simulink library "Autonomous_lib"  (R2023b)
settings: Solver=VariableStepAuto  StartTime=0.0  StopTime=10.0  RelTol=1e-3
settings Model: Creator=FIRSTMentor  LastModifiedBy=ander

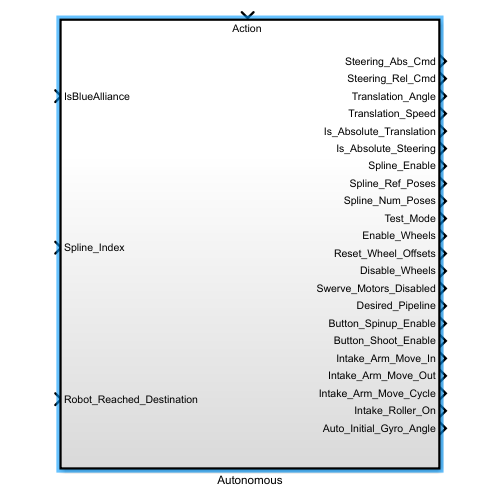
[thumbnail: Simulink's stored preview of the top-level diagram]
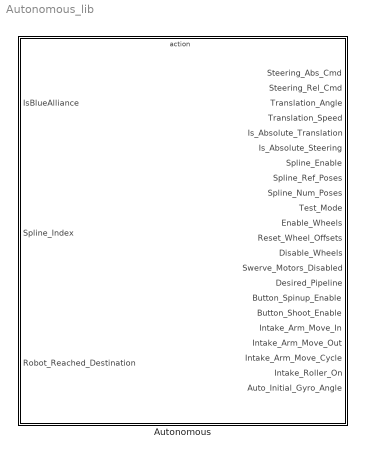
== system Autonomous_lib ==
  Autonomous : Subsystem  TreatAsAtomicUnit=on

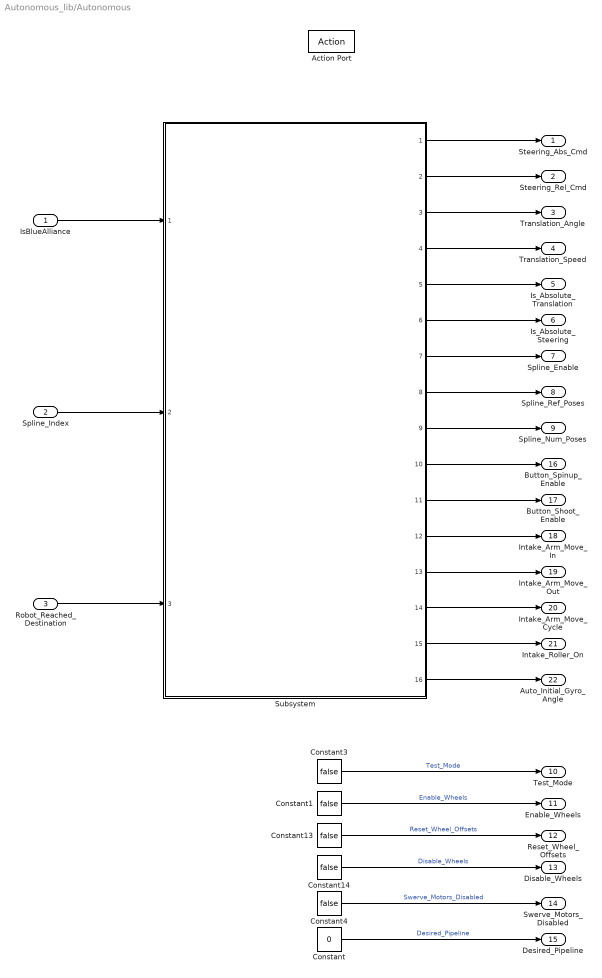
== system Autonomous_lib/Autonomous ==
  IsBlueAlliance : Inport
  Spline_Index : Inport  Port=2
  Robot_Reached_Destination : Inport  Port=3
  Action Port : ActionPort  InitializeStates=reset
  Constant : Constant  Value=0  OutDataTypeStr=uint8
  Constant{1,3..4,13..14} (5 alike) : Constant  Value=false  OutDataTypeStr=boolean
  Subsystem : Subsystem  ReferencedSubsystem=Autonomous_sub
  Steering_Abs_Cmd : Outport
  Steering_Rel_Cmd : Outport  Port=2
  Translation_Angle : Outport  Port=3
  Translation_Speed : Outport  Port=4
  Is_Absolute_Translation : Outport  Port=5
  Is_Absolute_Steering : Outport  Port=6
  Spline_Enable : Outport  Port=7
  Spline_Ref_Poses : Outport  Port=8
  Spline_Num_Poses : Outport  Port=9
  Test_Mode : Outport  Port=10
  Enable_Wheels : Outport  Port=11
  Reset_Wheel_Offsets : Outport  Port=12
  Disable_Wheels : Outport  Port=13
  Swerve_Motors_Disabled : Outport  Port=14
  Desired_Pipeline : Outport  Port=15
  Button_Spinup_Enable : Outport  Port=16
  Button_Shoot_Enable : Outport  Port=17
  Intake_Arm_Move_In : Outport  Port=18
  Intake_Arm_Move_Out : Outport  Port=19
  Intake_Arm_Move_Cycle : Outport  Port=20
  Intake_Roller_On : Outport  Port=21
  Auto_Initial_Gyro_Angle : Outport  Port=22
  wires:
  Constant3/1 -> Test_Mode/1  "Test_Mode"
  Constant14/1 -> Disable_Wheels/1  "Disable_Wheels"
  Constant13/1 -> Reset_Wheel_Offsets/1  "Reset_Wheel_Offsets"
  Constant4/1 -> Swerve_Motors_Disabled/1  "Swerve_Motors_Disabled"
  Constant1/1 -> Enable_Wheels/1  "Enable_Wheels"
  IsBlueAlliance/1 -> Subsystem/1
  Subsystem/1 -> Steering_Abs_Cmd/1
  Subsystem/2 -> Steering_Rel_Cmd/1
  Subsystem/3 -> Translation_Angle/1
  Subsystem/4 -> Translation_Speed/1
  Subsystem/5 -> Is_Absolute_Translation/1
  Subsystem/6 -> Is_Absolute_Steering/1
  Subsystem/7 -> Spline_Enable/1
  Subsystem/8 -> Spline_Ref_Poses/1
  Subsystem/9 -> Spline_Num_Poses/1
  Robot_Reached_Destination/1 -> Subsystem/3
  Constant/1 -> Desired_Pipeline/1  "Desired_Pipeline"
  Subsystem/10 -> Button_Spinup_Enable/1
  Subsystem/11 -> Button_Shoot_Enable/1
  Subsystem/12 -> Intake_Arm_Move_In/1
  Subsystem/13 -> Intake_Arm_Move_Out/1
  Subsystem/14 -> Intake_Arm_Move_Cycle/1
  Subsystem/15 -> Intake_Roller_On/1
  Spline_Index/1 -> Subsystem/2
  Subsystem/16 -> Auto_Initial_Gyro_Angle/1
